simulink model "ecu_mucur"  (R2026a)
settings: Solver=FixedStepDiscrete  StopTime=10  FixedStep=0.001  SampleTimeConstraint=STIndependent
Description:
  | Metering valve current loop. Source of truth for firmware/gen/ecu_mucur.
settings Model: Creator=jj1001000  LastModifiedBy=jj1001000
settings OptimizationCC: DefaultUnderspecifiedDataType=single
settings DebuggingCC: ParameterPrecisionLossMsg=none
settings HardwareCC: ProdLargestAtomicInteger=Long  ProdLargestAtomicFloat=Double  ProdHWDeviceType=ARM Compatible->ARM Cortex-M
settings RTWCC: SystemTargetFile=ert.tlc  GenCodeOnly=on  Description=Embedded Coder
settings ERTTargetCC: UtilityFuncGeneration=Shared location  IncludeMdlTerminateFcn=off  CodeInterfacePackaging=Reusable function  SupportNonFinite=off

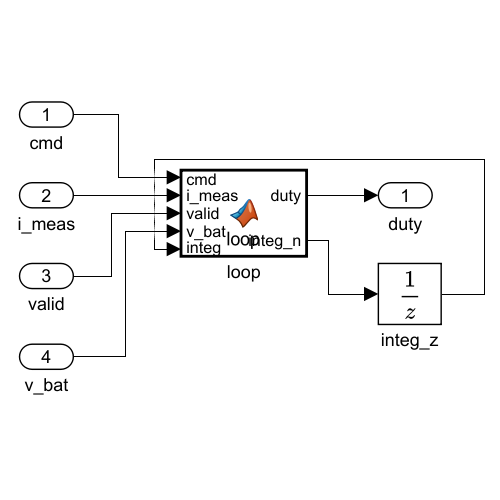
[thumbnail: Simulink's stored preview of the top-level diagram]
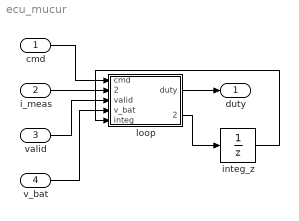
== system ecu_mucur ==
  cmd : Inport  OutDataTypeStr=single
  i_meas : Inport  Port=2  OutDataTypeStr=single
  valid : Inport  Port=3  OutDataTypeStr=uint8
  v_bat : Inport  Port=4  OutDataTypeStr=single
  integ_z : UnitDelay  SampleTime=-1
  loop : MATLAB Function  TreatAsAtomicUnit=on
  duty : Outport  OutDataTypeStr=single
  wires:
  cmd/1 -> loop/1(cmd)
  v_bat/1 -> loop/4(v_bat)
  valid/1 -> loop/3(valid)
  i_meas/1 -> loop/2(i_meas)
  loop/1(duty) -> duty/1
  loop/2(integ_n) -> integ_z/1
  integ_z/1 -> loop/5(integ)

== matlab function ecu_mucur/loop ==
  data: cmd input single; duty output single; i_meas input single; valid input uint8; v_bat input single; integ input single; integ_n output single
function [duty, integ_n] = loop(cmd, i_meas, valid, v_bat, integ)
%#codegen
if v_bat >= single(6) && v_bat <= single(18)
    vb = v_bat;
else
    vb = single(13.5);                       % no plausible reading: nominal
end
ff = cmd * (single(6.75) / vb);               % a nominal coil carries cmd * MU_I_FULL
if valid == 0
    integ_n = single(0);
    duty = sat(ff, single(0), single(1));
    return
end
err = cmd - i_meas / single(1.79999995);   % in units of the full current
out = ff + integ + single(0.100000001) * err;
integ_n = integ;
if ~((out >= single(1) && err > single(0)) || (out <= single(0) && err < single(0)))
    integ_n = sat(integ + single(10) * err * single(0.00100000005), single(-0.5), single(0.5));
end
duty = sat(ff + integ_n + single(0.100000001) * err, single(0), single(1));
end

function y = sat(x, lo, hi)
if x < lo
    y = lo;
elseif x > hi
    y = hi;
else
    y = x;
end
end
